simulink model "hrg_wa_v10_piezo"  (R2025a)
settings: Solver=FixedStepDiscrete  StartTime=0.0  StopTime=p.duration  FixedStep=p.Ts  RelTol=1e-3
model workspace (MAT data in the model file):
  Ad = [0.987688405123 5.68131323291e-08 -982.899001209 0.00680633562577 0 0 9.43869957356 -6.28544743895e-05 1136.68118394 -0.00505246365641 621.709647352 -0.00231548842692 ... (144 elements, 12x12)]
  Bd = [9.77654274822e-12  3.57356707517e-17; -3.57356707518e-17  9.77654274823e-12; 1.07045456936e-06  5.40868372992e-12; -5.40868372992e-12  1.07045456936e-06; 0.71349520314  0; 0  0.71349520314; -1.000960045e-08  -4.85539211802e-14; 4.85539211802e-14  -1.000960045e-08; -8.77502484995e-07  -3.08787328803e-12; 3.08787328803e-12  -8.77502484995e-07; -4.16709269638e-07  -1.25256309993e-12; 1.25256309993e-12  -4.16709269638e-07]
  p.synthetic = 1
  p.f0 = 1000
  p.mass = 0.0001
  p.Q = 10000
  p.B = 0.276990961962
  p.amp = 1e-06
  p.initial_amp = 3e-07
  p.alpha0 = 0.4
  p.Omega = 0.5
  p.Ts = 2.5e-05
  p.duration = 1
  p.Tc = 0.001
  p.Cf = 1e-10
  p.Rf = 1000000000
  p.Cs = 1e-09
  p.Rs = 1000
  p.theta_s = 1e-05
  p.theta_d = 1e-05
  p.Cds = 0
  p.driver_tau = 2e-05
  p.afe_bw = 20000
  p.adc_span = 2
  p.adc_bits = 20
  p.dac_span = 2
  p.dac_bits = 18
  p.vmax = 1
  p.gain_y = 1
  p.drive_y = 1
  p.calibrate = 1
  p.compensate_drive = 1
  p.agc_bw = 5
  p.quad_bw = 4
  p.pll_gain = 30
  p.max_detune = 30
  p.noise_rms = 0
  p.seed = 29
  p.damping_delta = 0
  p.split_hz = 0
  p.phase_y = 0
  x0 = [2.76318298201e-07; 1.16825502693e-07; 0; 0; 0; 0; 0; 0; 0; 0; 0; 0]
Description:
  | V10 synthetic piezo carrier closed loop. State pairs: q,velocity,driver voltage,sensor voltage,charge amplifier,AFE. Equations and limitations in docs.
settings Model: Creator=11725  LastModifiedBy=11725

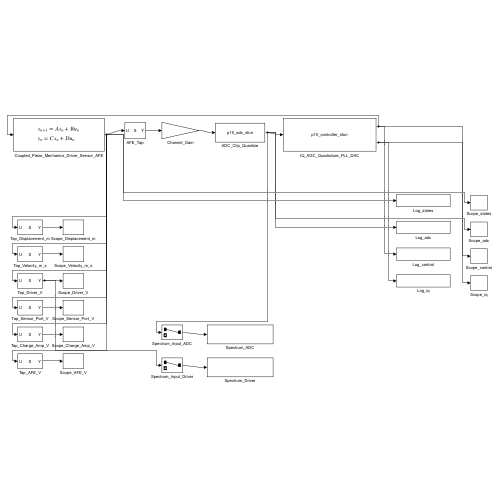
[thumbnail: Simulink's stored preview of the top-level diagram]
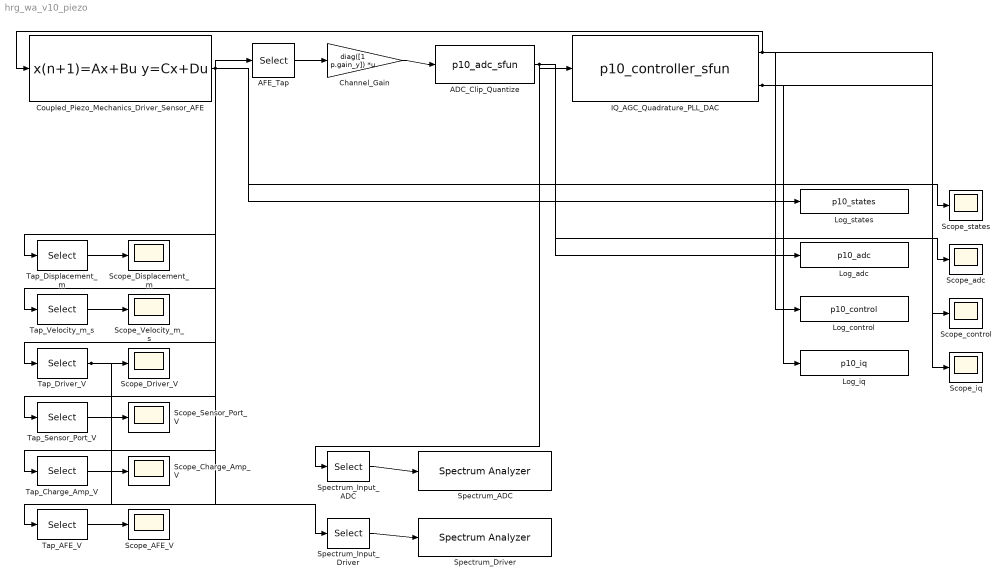
== system hrg_wa_v10_piezo ==
  ADC_Clip_Quantize : M-S-Function  FunctionName=p10_adc_sfun  Parameters=p
  AFE_Tap : Selector  InputPortWidth=12  IndexOptions=Index vector (dialog)  Indices=[11 12]  OutputSizes=1
  Channel_Gain : Gain  Gain=diag([1 p.gain_y])  Multiplication=Matrix(K*u)
  Coupled_Piezo_Mechanics_Driver_Sensor_AFE : DiscreteStateSpace  A=Ad  B=Bd  C=eye(12)  D=zeros(12,2)  InitialCondition=x0  SampleTime=p.Ts
  IQ_AGC_Quadrature_PLL_DAC : M-S-Function  FunctionName=p10_controller_sfun  Parameters=p
  Log_adc : ToWorkspace  VariableName=p10_adc  SaveFormat=Timeseries  SampleTime=-1
  Log_control : ToWorkspace  VariableName=p10_control  SaveFormat=Timeseries  SampleTime=-1
  Log_iq : ToWorkspace  VariableName=p10_iq  SaveFormat=Timeseries  SampleTime=-1
  Log_states : ToWorkspace  VariableName=p10_states  SaveFormat=Timeseries  SampleTime=-1
  Scope_AFE_V : Scope
  Scope_Charge_Amp_V : Scope
  Scope_Displacement_m : Scope
  Scope_Driver_V : Scope
  Scope_Sensor_Port_V : Scope
  Scope_Velocity_m_s : Scope
  Scope_adc : Scope
  Scope_control : Scope
  Scope_iq : Scope
  Scope_states : Scope
  Spectrum_ADC : SpectrumAnalyzer  SampleRateSource=Property  SampleRate=40000  WindowInvariantSamplesPerUpdate=on  SpectrumUnits=dBV
      settings: OpenAtSimulationStart=off
  Spectrum_Driver : SpectrumAnalyzer  SampleRateSource=Property  SampleRate=40000  WindowInvariantSamplesPerUpdate=on  SpectrumUnits=dBV
      settings: OpenAtSimulationStart=off
  Spectrum_Input_ADC : Selector  InputPortWidth=2  IndexOptions=Index vector (dialog)  Indices=1  OutputSizes=1
  Spectrum_Input_Driver : Selector  InputPortWidth=2  IndexOptions=Index vector (dialog)  Indices=1  OutputSizes=1
  Tap_AFE_V : Selector  InputPortWidth=12  IndexOptions=Index vector (dialog)  Indices=[11 12]  OutputSizes=1
  Tap_Charge_Amp_V : Selector  InputPortWidth=12  IndexOptions=Index vector (dialog)  Indices=[9 10]  OutputSizes=1
  Tap_Displacement_m : Selector  InputPortWidth=12  IndexOptions=Index vector (dialog)  Indices=[1 2]  OutputSizes=1
  Tap_Driver_V : Selector  InputPortWidth=12  IndexOptions=Index vector (dialog)  Indices=[5 6]  OutputSizes=1
  Tap_Sensor_Port_V : Selector  InputPortWidth=12  IndexOptions=Index vector (dialog)  Indices=[7 8]  OutputSizes=1
  Tap_Velocity_m_s : Selector  InputPortWidth=12  IndexOptions=Index vector (dialog)  Indices=[3 4]  OutputSizes=1
  wires:
  Coupled_Piezo_Mechanics_Driver_Sensor_AFE/1 -> AFE_Tap/1, Log_states/1, Scope_states/1, Tap_Displacement_m/1, Tap_Velocity_m_s/1, Tap_Driver_V/1, Tap_Sensor_Port_V/1, Tap_Charge_Amp_V/1, Tap_AFE_V/1
  AFE_Tap/1 -> Channel_Gain/1
  Channel_Gain/1 -> ADC_Clip_Quantize/1
  ADC_Clip_Quantize/1 -> IQ_AGC_Quadrature_PLL_DAC/1, Log_adc/1, Scope_adc/1, Spectrum_Input_ADC/1
  IQ_AGC_Quadrature_PLL_DAC/1 -> Coupled_Piezo_Mechanics_Driver_Sensor_AFE/1, Log_control/1, Scope_control/1
  IQ_AGC_Quadrature_PLL_DAC/2 -> Log_iq/1, Scope_iq/1
  Tap_Displacement_m/1 -> Scope_Displacement_m/1
  Tap_Velocity_m_s/1 -> Scope_Velocity_m_s/1
  Tap_Driver_V/1 -> Scope_Driver_V/1, Spectrum_Input_Driver/1
  Tap_Sensor_Port_V/1 -> Scope_Sensor_Port_V/1
  Tap_Charge_Amp_V/1 -> Scope_Charge_Amp_V/1
  Tap_AFE_V/1 -> Scope_AFE_V/1
  Spectrum_Input_ADC/1 -> Spectrum_ADC/1
  Spectrum_Input_Driver/1 -> Spectrum_Driver/1
